simulink model "SDA_PL_Harness_2025b"  (R2025b)
settings: Solver=FixedStepDiscrete  StartTime=0.0  StopTime=inf  FixedStep=1e-8  RelTol=1e-3
PreLoadFcn:
  | addpath('C:\Users\Cheng\Documents\MasterThesis\Model_2025b\Harness');
InitFcn:
  | setup_sda_harness_workspace_2025b;
undefined symbols (not defined in the file or in its folder): sdaHarnessAbsTol, sdaHarnessCaseLimit, sdaHarnessData, sdaHarnessRelTol
(part 1 of 2)
settings Model: DataDictionary=FOC_params.sldd  Creator=Cheng  LastModifiedBy=Cheng

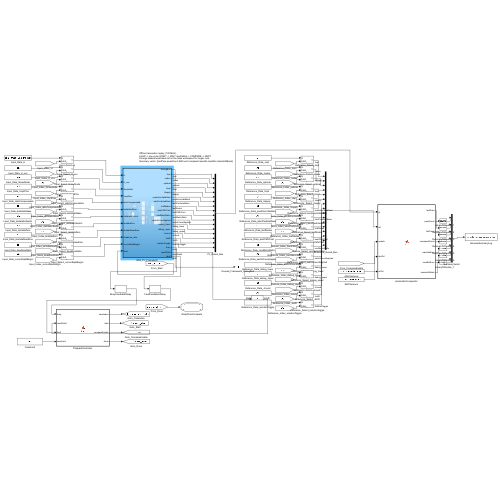
[thumbnail: Simulink's stored preview of the top-level diagram]
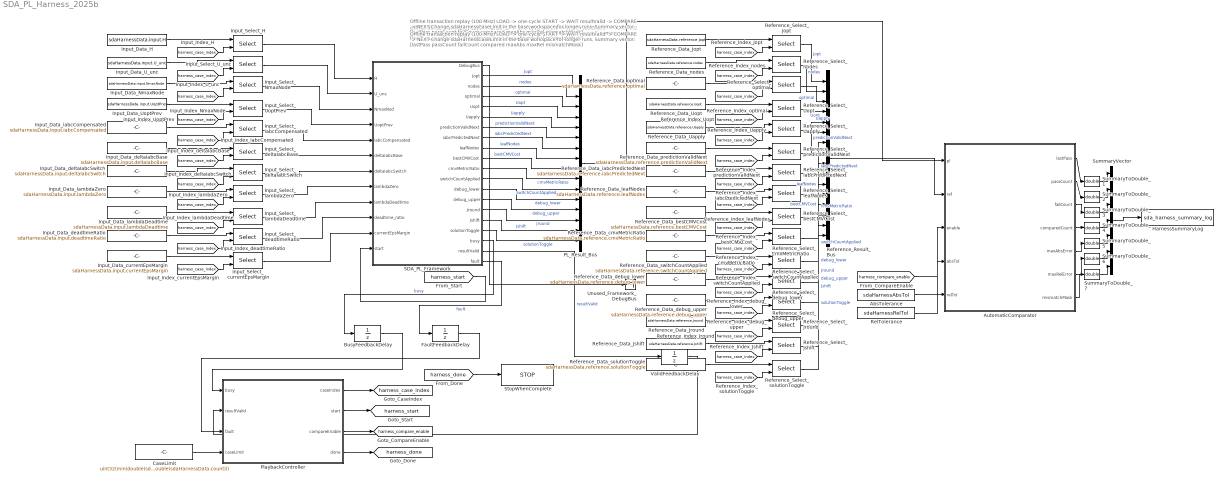
== system SDA_PL_Harness_2025b ==
  note: Offline transaction replay (100 MHz)
      | LOAD -> one-cycle START -> WAIT resultValid -> COMPARE -> NEXT
      | Change sdaHarnessCaseLimit in the base workspace for longer runs.
      | Summary vector: [lastPass passCount failCount compared maxAbs maxRel mismatchMask]
  note: Offline transaction replay (100 MHz)
      | LOAD -> one-cycle START -> WAIT resultValid -> COMPARE -> NEXT
      | Change sdaHarnessCaseLimit in the base workspace for longer runs.
      | Summary vector: [lastPass passCount failCount compared maxAbs maxRel mismatchMask]
  note: Offline transaction replay (100 MHz)
      | LOAD -> one-cycle START -> WAIT resultValid -> COMPARE -> NEXT
      | Change sdaHarnessCaseLimit in the base workspace for longer runs.
      | Summary vector: [lastPass passCount failCount compared maxAbs maxRel mismatchMask]
  note: Offline transaction replay (100 MHz)
      | LOAD -> one-cycle START -> WAIT resultValid -> COMPARE -> NEXT
      | Change sdaHarnessCaseLimit in the base workspace for longer runs.
      | Summary vector: [lastPass passCount failCount compared maxAbs maxRel mismatchMask]
  note: Offline transaction replay (100 MHz)
      | LOAD -> one-cycle START -> WAIT resultValid -> COMPARE -> NEXT
      | Change sdaHarnessCaseLimit in the base workspace for longer runs.
      | Summary vector: [lastPass passCount failCount compared maxAbs maxRel mismatchMask]
  note: Offline transaction replay (100 MHz)
      | LOAD -> one-cycle START -> WAIT resultValid -> COMPARE -> NEXT
      | Change sdaHarnessCaseLimit in the base workspace for longer runs.
      | Summary vector: [lastPass passCount failCount compared maxAbs maxRel mismatchMask]
  AbsTolerance : Constant  Value=sdaHarnessAbsTol
  AutomaticComparator : MATLAB Function  TreatAsAtomicUnit=on
  BusyFeedbackDelay : UnitDelay  InitialCondition=false  SampleTime=1e-8  HasFrameUpgradeWarning=on
  CaseLimit : Constant  Value=uint32(min(double(sdaHarnessCaseLimit),double(sdaHarnessData.count)))  OutDataTypeStr=uint32
  FaultFeedbackDelay : UnitDelay  InitialCondition=false  SampleTime=1e-8  HasFrameUpgradeWarning=on
  HarnessSummaryLog : ToWorkspace  VariableName=sda_harness_summary_log  SaveFormat=Timeseries  SampleTime=-1
  Input_Data_H : Constant  Value=sdaHarnessData.input.H
  Input_Data_NmaxNode : Constant  Value=sdaHarnessData.input.NmaxNode
  Input_Data_U_unc : Constant  Value=sdaHarnessData.input.U_unc
  Input_Data_UoptPrev : Constant  Value=sdaHarnessData.input.UoptPrev
  Input_Data_currentEpsMargin : Constant  Value=sdaHarnessData.input.currentEpsMargin
  Input_Data_deadtimeRatio : Constant  Value=sdaHarnessData.input.deadtimeRatio
  Input_Data_deltaIabcBase : Constant  Value=sdaHarnessData.input.deltaIabcBase
  Input_Data_deltaIabcSwitch : Constant  Value=sdaHarnessData.input.deltaIabcSwitch
  Input_Data_iabcCompensated : Constant  Value=sdaHarnessData.input.iabcCompensated
  Input_Data_lambdaDeadtime : Constant  Value=sdaHarnessData.input.lambdaDeadtime
  Input_Data_lambdaZero : Constant  Value=sdaHarnessData.input.lambdaZero
  Input_Select_H : Selector  NumberOfDimensions=3  InputPortWidth=3  IndexOptions=Select all,Select all,Index vector (port)  Indices=1,1,1  OutputSizes=1
  Input_Select_NmaxNode : Selector  NumberOfDimensions=2  InputPortWidth=3  IndexOptions=Index vector (dialog),Index vector (port)  Indices=1,1  OutputSizes=1
  Input_Select_U_unc : Selector  NumberOfDimensions=2  InputPortWidth=3  IndexOptions=Select all,Index vector (port)  Indices=1,1  OutputSizes=1
  Input_Select_UoptPrev : Selector  NumberOfDimensions=2  InputPortWidth=3  IndexOptions=Select all,Index vector (port)  Indices=1,1  OutputSizes=1
  Input_Select_currentEpsMargin : Selector  NumberOfDimensions=2  InputPortWidth=3  IndexOptions=Index vector (dialog),Index vector (port)  Indices=1,1  OutputSizes=1
  Input_Select_deadtimeRatio : Selector  NumberOfDimensions=2  InputPortWidth=3  IndexOptions=Index vector (dialog),Index vector (port)  Indices=1,1  OutputSizes=1
  Input_Select_deltaIabcBase : Selector  NumberOfDimensions=2  InputPortWidth=3  IndexOptions=Select all,Index vector (port)  Indices=1,1  OutputSizes=1
  Input_Select_deltaIabcSwitch : Selector  NumberOfDimensions=3  InputPortWidth=3  IndexOptions=Select all,Select all,Index vector (port)  Indices=1,1,1  OutputSizes=1
  Input_Select_iabcCompensated : Selector  NumberOfDimensions=2  InputPortWidth=3  IndexOptions=Select all,Index vector (port)  Indices=1,1  OutputSizes=1
  Input_Select_lambdaDeadtime : Selector  NumberOfDimensions=2  InputPortWidth=3  IndexOptions=Index vector (dialog),Index vector (port)  Indices=1,1  OutputSizes=1
  Input_Select_lambdaZero : Selector  NumberOfDimensions=2  InputPortWidth=3  IndexOptions=Index vector (dialog),Index vector (port)  Indices=1,1  OutputSizes=1
  PL_Result_Bus : BusCreator  Inputs=16  OutDataTypeStr=Bus: SdaComparisonResultBus
  PlaybackController : MATLAB Function  TreatAsAtomicUnit=on
  Reference_Data_Jopt : Constant  Value=sdaHarnessData.reference.Jopt
  Reference_Data_Jround : Constant  Value=sdaHarnessData.reference.Jround
  Reference_Data_Jshift : Constant  Value=sdaHarnessData.reference.Jshift
  Reference_Data_Uapply : Constant  Value=sdaHarnessData.reference.Uapply
  Reference_Data_Uopt : Constant  Value=sdaHarnessData.reference.Uopt
  Reference_Data_bestCMVCost : Constant  Value=sdaHarnessData.reference.bestCMVCost
  Reference_Data_cmvMetricRatio : Constant  Value=sdaHarnessData.reference.cmvMetricRatio
  Reference_Data_debug_lower : Constant  Value=sdaHarnessData.reference.debug_lower
  Reference_Data_debug_upper : Constant  Value=sdaHarnessData.reference.debug_upper
  Reference_Data_iabcPredictedNext : Constant  Value=sdaHarnessData.reference.iabcPredictedNext
  Reference_Data_leafNodes : Constant  Value=sdaHarnessData.reference.leafNodes
  Reference_Data_nodes : Constant  Value=sdaHarnessData.reference.nodes
  Reference_Data_optimal : Constant  Value=sdaHarnessData.reference.optimal
  Reference_Data_predictionValidNext : Constant  Value=sdaHarnessData.reference.predictionValidNext
  Reference_Data_solutionToggle : Constant  Value=sdaHarnessData.reference.solutionToggle
  Reference_Data_switchCountApplied : Constant  Value=sdaHarnessData.reference.switchCountApplied
  Reference_Result_Bus : BusCreator  Inputs=16  OutDataTypeStr=Bus: SdaComparisonResultBus
  Reference_Select_Jopt : Selector  NumberOfDimensions=2  InputPortWidth=3  IndexOptions=Index vector (dialog),Index vector (port)  Indices=1,1  OutputSizes=1
  Reference_Select_Jround : Selector  NumberOfDimensions=2  InputPortWidth=3  IndexOptions=Index vector (dialog),Index vector (port)  Indices=1,1  OutputSizes=1
  Reference_Select_Jshift : Selector  NumberOfDimensions=2  InputPortWidth=3  IndexOptions=Index vector (dialog),Index vector (port)  Indices=1,1  OutputSizes=1
  Reference_Select_Uapply : Selector  NumberOfDimensions=2  InputPortWidth=3  IndexOptions=Select all,Index vector (port)  Indices=1,1  OutputSizes=1
  Reference_Select_Uopt : Selector  NumberOfDimensions=2  InputPortWidth=3  IndexOptions=Select all,Index vector (port)  Indices=1,1  OutputSizes=1
  Reference_Select_bestCMVCost : Selector  NumberOfDimensions=2  InputPortWidth=3  IndexOptions=Index vector (dialog),Index vector (port)  Indices=1,1  OutputSizes=1
  Reference_Select_cmvMetricRatio : Selector  NumberOfDimensions=2  InputPortWidth=3  IndexOptions=Index vector (dialog),Index vector (port)  Indices=1,1  OutputSizes=1
  Reference_Select_debug_lower : Selector  NumberOfDimensions=2  InputPortWidth=3  IndexOptions=Select all,Index vector (port)  Indices=1,1  OutputSizes=1
  Reference_Select_debug_upper : Selector  NumberOfDimensions=2  InputPortWidth=3  IndexOptions=Select all,Index vector (port)  Indices=1,1  OutputSizes=1
  Reference_Select_iabcPredictedNext : Selector  NumberOfDimensions=2  InputPortWidth=3  IndexOptions=Select all,Index vector (port)  Indices=1,1  OutputSizes=1
  Reference_Select_leafNodes : Selector  NumberOfDimensions=2  InputPortWidth=3  IndexOptions=Index vector (dialog),Index vector (port)  Indices=1,1  OutputSizes=1
  Reference_Select_nodes : Selector  NumberOfDimensions=2  InputPortWidth=3  IndexOptions=Index vector (dialog),Index vector (port)  Indices=1,1  OutputSizes=1
  Reference_Select_optimal : Selector  NumberOfDimensions=2  InputPortWidth=3  IndexOptions=Index vector (dialog),Index vector (port)  Indices=1,1  OutputSizes=1
  Reference_Select_predictionValidNext : Selector  NumberOfDimensions=2  InputPortWidth=3  IndexOptions=Index vector (dialog),Index vector (port)  Indices=1,1  OutputSizes=1
  Reference_Select_solutionToggle : Selector  NumberOfDimensions=2  InputPortWidth=3  IndexOptions=Index vector (dialog),Index vector (port)  Indices=1,1  OutputSizes=1
  Reference_Select_switchCountApplied : Selector  NumberOfDimensions=2  InputPortWidth=3  IndexOptions=Index vector (dialog),Index vector (port)  Indices=1,1  OutputSizes=1
  RelTolerance : Constant  Value=sdaHarnessRelTol
  SDA_PL_Framework : Subsystem  TreatAsAtomicUnit=on
  StopWhenComplete : Stop
  SummaryToDouble_{1..7} (7 alike) : DataTypeConversion  OutDataTypeStr=double  SaturateOnIntegerOverflow=off  RndMeth=Floor
  SummaryVector : Mux  Inputs=7
  Unused_Framework_DebugBus : Terminator
  ValidFeedbackDelay : UnitDelay  InitialCondition=false  SampleTime=1e-8  HasFrameUpgradeWarning=on
  tag scope: harness_case_index=global, harness_compare_enable=global, harness_done=global, harness_start=global
  wires:
  CaseLimit/1 -> PlaybackController/4(caseLimit)
  PlaybackController/1(caseIndex) -> [harness_case_index]
  PlaybackController/2(start) -> [harness_start]
  PlaybackController/3(compareEnable) -> [harness_compare_enable]
  PlaybackController/4(done) -> [harness_done]
  Input_Data_H/1 -> Input_Select_H/1
  [harness_case_index] -> Input_Select_H/2
  Input_Data_U_unc/1 -> Input_Select_U_unc/1
  [harness_case_index] -> Input_Select_U_unc/2
  Input_Data_NmaxNode/1 -> Input_Select_NmaxNode/1
  [harness_case_index] -> Input_Select_NmaxNode/2
  Input_Data_UoptPrev/1 -> Input_Select_UoptPrev/1
  [harness_case_index] -> Input_Select_UoptPrev/2
  Input_Data_iabcCompensated/1 -> Input_Select_iabcCompensated/1
  [harness_case_index] -> Input_Select_iabcCompensated/2
  Input_Data_deltaIabcBase/1 -> Input_Select_deltaIabcBase/1
  [harness_case_index] -> Input_Select_deltaIabcBase/2
  Input_Data_deltaIabcSwitch/1 -> Input_Select_deltaIabcSwitch/1
  [harness_case_index] -> Input_Select_deltaIabcSwitch/2
  Input_Data_lambdaZero/1 -> Input_Select_lambdaZero/1
  [harness_case_index] -> Input_Select_lambdaZero/2
  Input_Data_lambdaDeadtime/1 -> Input_Select_lambdaDeadtime/1
  [harness_case_index] -> Input_Select_lambdaDeadtime/2
  Input_Data_deadtimeRatio/1 -> Input_Select_deadtimeRatio/1
  [harness_case_index] -> Input_Select_deadtimeRatio/2
  Input_Data_currentEpsMargin/1 -> Input_Select_currentEpsMargin/1
  [harness_case_index] -> Input_Select_currentEpsMargin/2
  Reference_Data_Jopt/1 -> Reference_Select_Jopt/1
  [harness_case_index] -> Reference_Select_Jopt/2
  Reference_Data_nodes/1 -> Reference_Select_nodes/1
  [harness_case_index] -> Reference_Select_nodes/2
  Reference_Data_optimal/1 -> Reference_Select_optimal/1
  [harness_case_index] -> Reference_Select_optimal/2
  Reference_Data_Uopt/1 -> Reference_Select_Uopt/1
  [harness_case_index] -> Reference_Select_Uopt/2
  Reference_Data_Uapply/1 -> Reference_Select_Uapply/1
  [harness_case_index] -> Reference_Select_Uapply/2
  Reference_Data_predictionValidNext/1 -> Reference_Select_predictionValidNext/1
  [harness_case_index] -> Reference_Select_predictionValidNext/2
  Reference_Data_iabcPredictedNext/1 -> Reference_Select_iabcPredictedNext/1
  [harness_case_index] -> Reference_Select_iabcPredictedNext/2
  Reference_Data_leafNodes/1 -> Reference_Select_leafNodes/1
  [harness_case_index] -> Reference_Select_leafNodes/2
  Reference_Data_bestCMVCost/1 -> Reference_Select_bestCMVCost/1
  [harness_case_index] -> Reference_Select_bestCMVCost/2
  Reference_Data_cmvMetricRatio/1 -> Reference_Select_cmvMetricRatio/1
  [harness_case_index] -> Reference_Select_cmvMetricRatio/2
  Reference_Data_switchCountApplied/1 -> Reference_Select_switchCountApplied/1
  [harness_case_index] -> Reference_Select_switchCountApplied/2
  Reference_Data_debug_lower/1 -> Reference_Select_debug_lower/1
  [harness_case_index] -> Reference_Select_debug_lower/2
  Reference_Data_debug_upper/1 -> Reference_Select_debug_upper/1
  [harness_case_index] -> Reference_Select_debug_upper/2
  Reference_Data_Jround/1 -> Reference_Select_Jround/1
  [harness_case_index] -> Reference_Select_Jround/2
  Reference_Data_Jshift/1 -> Reference_Select_Jshift/1
  [harness_case_index] -> Reference_Select_Jshift/2
  Reference_Data_solutionToggle/1 -> Reference_Select_solutionToggle/1
  [harness_case_index] -> Reference_Select_solutionToggle/2
  Input_Select_H/1 -> SDA_PL_Framework/1(H)
  Input_Select_U_unc/1 -> SDA_PL_Framework/2(U_unc)
  Input_Select_NmaxNode/1 -> SDA_PL_Framework/3(NmaxNod)
  Input_Select_UoptPrev/1 -> SDA_PL_Framework/4(UoptPrev)
  Input_Select_iabcCompensated/1 -> SDA_PL_Framework/5(iabcCompensated)
  Input_Select_deltaIabcBase/1 -> SDA_PL_Framework/6(deltaIabcBase)
  Input_Select_deltaIabcSwitch/1 -> SDA_PL_Framework/7(deltaIabcSwitch)
  Input_Select_lambdaZero/1 -> SDA_PL_Framework/8(lambdaZero)
  Input_Select_lambdaDeadtime/1 -> SDA_PL_Framework/9(lambdaDeadtime)
  Input_Select_deadtimeRatio/1 -> SDA_PL_Framework/10(deadtime_ratio)
  Input_Select_currentEpsMargin/1 -> SDA_PL_Framework/11(currentEpsMargin)
  [harness_start] -> SDA_PL_Framework/12(start)
  SDA_PL_Framework/2(Jopt) -> PL_Result_Bus/1  "Jopt"
  Reference_Select_Jopt/1 -> Reference_Result_Bus/1  "Jopt"
  SDA_PL_Framework/3(nodes) -> PL_Result_Bus/2  "nodes"
  Reference_Select_nodes/1 -> Reference_Result_Bus/2  "nodes"
  SDA_PL_Framework/4(optimal) -> PL_Result_Bus/3  "optimal"
  Reference_Select_optimal/1 -> Reference_Result_Bus/3  "optimal"
  SDA_PL_Framework/5(Uopt) -> PL_Result_Bus/4  "Uopt"
  Reference_Select_Uopt/1 -> Reference_Result_Bus/4  "Uopt"
  SDA_PL_Framework/6(Uapply) -> PL_Result_Bus/5  "Uapply"
  Reference_Select_Uapply/1 -> Reference_Result_Bus/5  "Uapply"
  SDA_PL_Framework/7(predictionValidNext) -> PL_Result_Bus/6  "predictionValidNext"
  Reference_Select_predictionValidNext/1 -> Reference_Result_Bus/6  "predictionValidNext"
  SDA_PL_Framework/8(iabcPredictedNext) -> PL_Result_Bus/7  "iabcPredictedNext"
  Reference_Select_iabcPredictedNext/1 -> Reference_Result_Bus/7  "iabcPredictedNext"
  SDA_PL_Framework/9(leafNodes) -> PL_Result_Bus/8  "leafNodes"
  Reference_Select_leafNodes/1 -> Reference_Result_Bus/8  "leafNodes"
  SDA_PL_Framework/10(bestCMVCost) -> PL_Result_Bus/9  "bestCMVCost"
  Reference_Select_bestCMVCost/1 -> Reference_Result_Bus/9  "bestCMVCost"
  SDA_PL_Framework/11(cmvMetricRatio) -> PL_Result_Bus/10  "cmvMetricRatio"
  Reference_Select_cmvMetricRatio/1 -> Reference_Result_Bus/10  "cmvMetricRatio"
  SDA_PL_Framework/12(switchCountApplied) -> PL_Result_Bus/11  "switchCountApplied"
  Reference_Select_switchCountApplied/1 -> Reference_Result_Bus/11  "switchCountApplied"
  SDA_PL_Framework/13(debug_lower) -> PL_Result_Bus/12  "debug_lower"
  Reference_Select_debug_lower/1 -> Reference_Result_Bus/12  "debug_lower"
  SDA_PL_Framework/14(debug_upper) -> PL_Result_Bus/13  "debug_upper"
  Reference_Select_debug_upper/1 -> Reference_Result_Bus/13  "debug_upper"
  SDA_PL_Framework/15(Jround) -> PL_Result_Bus/14  "Jround"
  Reference_Select_Jround/1 -> Reference_Result_Bus/14  "Jround"
  SDA_PL_Framework/16(Jshift) -> PL_Result_Bus/15  "Jshift"
  Reference_Select_Jshift/1 -> Reference_Result_Bus/15  "Jshift"
  SDA_PL_Framework/17(solutionToggle) -> PL_Result_Bus/16  "solutionToggle"
  Reference_Select_solutionToggle/1 -> Reference_Result_Bus/16  "solutionToggle"
  PL_Result_Bus/1 -> AutomaticComparator/1(pl)
  Reference_Result_Bus/1 -> AutomaticComparator/2(ref)
  [harness_compare_enable] -> AutomaticComparator/3(enable)
  AbsTolerance/1 -> AutomaticComparator/4(absTol)
  RelTolerance/1 -> AutomaticComparator/5(relTol)
  AutomaticComparator/1(lastPass) -> SummaryToDouble_1/1
  SummaryToDouble_1/1 -> SummaryVector/1
  AutomaticComparator/2(passCount) -> SummaryToDouble_2/1
  SummaryToDouble_2/1 -> SummaryVector/2
  AutomaticComparator/3(failCount) -> SummaryToDouble_3/1
  SummaryToDouble_3/1 -> SummaryVector/3
  AutomaticComparator/4(comparedCount) -> SummaryToDouble_4/1
  SummaryToDouble_4/1 -> SummaryVector/4
  AutomaticComparator/5(maxAbsError) -> SummaryToDouble_5/1
  SummaryToDouble_5/1 -> SummaryVector/5
  AutomaticComparator/6(maxRelError) -> SummaryToDouble_6/1
  SummaryToDouble_6/1 -> SummaryVector/6
  AutomaticComparator/7(mismatchMask) -> SummaryToDouble_7/1
  SummaryToDouble_7/1 -> SummaryVector/7
  SummaryVector/1 -> HarnessSummaryLog/1
  [harness_done] -> StopWhenComplete/1
  SDA_PL_Framework/18(busy) -> BusyFeedbackDelay/1  "busy"
  BusyFeedbackDelay/1 -> PlaybackController/1(busy)
  SDA_PL_Framework/19(resultValid) -> ValidFeedbackDelay/1  "resultValid"
  ValidFeedbackDelay/1 -> PlaybackController/2(resultValid)
  SDA_PL_Framework/20(fault) -> FaultFeedbackDelay/1  "fault"
  FaultFeedbackDelay/1 -> PlaybackController/3(fault)
  SDA_PL_Framework/1(DebugBus) -> Unused_Framework_DebugBus/1

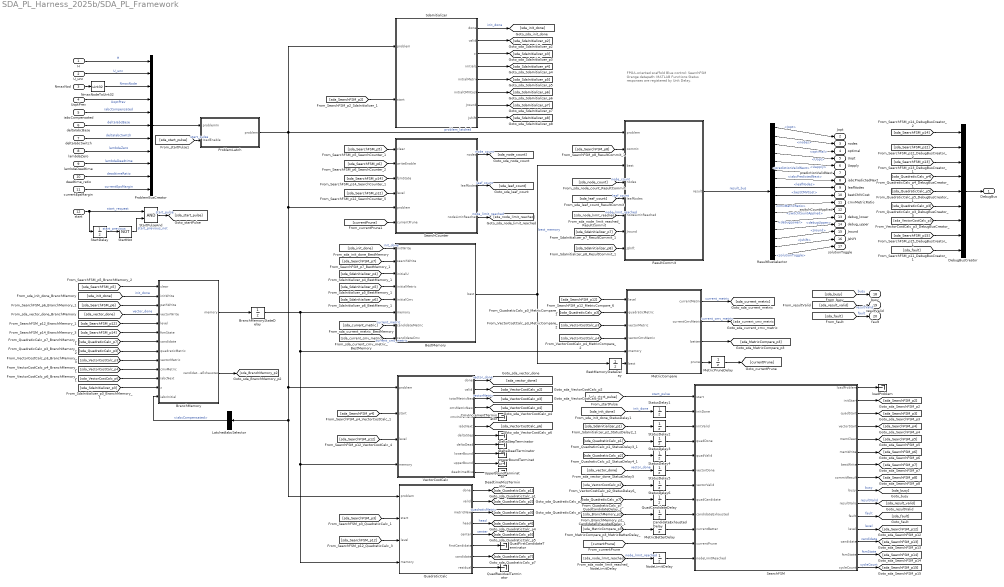
== system SDA_PL_Harness_2025b/SDA_PL_Framework ==
  note: FPGA-oriented scaffold
      | Blue control: SearchFSM
      | Orange datapath: MATLAB Functions
      | Status responses are registered by Unit Delay.
  H : Inport
  U_unc : Inport  Port=2
  NmaxNod : Inport  Port=3
  UoptPrev : Inport  Port=4
  iabcCompensated : Inport  Port=5
  deltaIabcBase : Inport  Port=6
  deltaIabcSwitch : Inport  Port=7
  lambdaZero : Inport  Port=8
  lambdaDeadtime : Inport  Port=9
  deadtime_ratio : Inport  Port=10
  currentEpsMargin : Inport  Port=11
  start : Inport  Port=12  OutDataTypeStr=boolean
  BestMemory : MATLAB Function  TreatAsAtomicUnit=on
  BestMemoryStateDelay : UnitDelay  SampleTime=-1
  BranchMemory : MATLAB Function  TreatAsAtomicUnit=on
  BranchMemoryStateDelay : UnitDelay  SampleTime=-1
  CandidateExhaustedDelay : UnitDelay  InitialCondition=false  SampleTime=-1
  CmvIncrementTerminator : Terminator
  DeadtimeMissTerminator : Terminator
  DebugBusCreator : BusCreator  Inputs=9  OutDataTypeStr=Bus: SdaDebugBus
  DeltaDeadTerminator : Terminator
  DeltaStepTerminator : Terminator
  LatchedIabcSelector : BusSelector  OutputSignals=iabcCompensated
  LowerBoundTerminator : Terminator
  MetricBetterDelay : UnitDelay  InitialCondition=false  SampleTime=-1
  MetricCompare : MATLAB Function  TreatAsAtomicUnit=on
  MetricPruneDelay : UnitDelay  InitialCondition=false  SampleTime=-1
  NmaxNodeToUint32 : DataTypeConversion  OutDataTypeStr=uint32  SaturateOnIntegerOverflow=off  RndMeth=Floor
  NodeLimitDelay : UnitDelay  InitialCondition=false  SampleTime=-1
  ProblemBusCreator : BusCreator  Inputs=11  OutDataTypeStr=Bus: SdaProblemBus
  ProblemLatch : MATLAB Function  TreatAsAtomicUnit=on
  QuadCandidateDelay : UnitDelay  InitialCondition=false  SampleTime=-1
  QuadFirstCandidateTerminator : Terminator
  QuadResidualTerminator : Terminator
  QuadraticCalc : MATLAB Function  TreatAsAtomicUnit=on
  ResultBusSelector : BusSelector  OutputSignals=Jopt,nodes,optimal,Uopt,Uapply,predictionValidNext,iabcPredictedNext,leafNodes,bestCMVCost,cmvMetricRatio,switchCountApplied,debugLower,debugUpper,Jround,Jshift,solutionToggle
  ResultCommit : MATLAB Function  TreatAsAtomicUnit=on
  SdaInitializer : MATLAB Function  TreatAsAtomicUnit=on
  SearchCounter : MATLAB Function  TreatAsAtomicUnit=on
  SearchFSM : Stateflow chart  TreatAsAtomicUnit=on
  StartDelay : UnitDelay  InitialCondition=false  SampleTime=-1  HasFrameUpgradeWarning=on
  StartNot : Logic  Operator=NOT  AllPortsSameDT=off  OutDataTypeStr=boolean
  StartPulseAnd : Logic  AllPortsSameDT=off  OutDataTypeStr=boolean
  StatusDelay{1..6} (6 alike) : UnitDelay  InitialCondition=false  SampleTime=-1
  UpperBoundTerminator : Terminator
  VectorCostCalc : MATLAB Function  TreatAsAtomicUnit=on
  loadProblem : Terminator
  DebugBus : Outport  OutDataTypeStr=Bus: SdaDebugBus
  Jopt : Outport  Port=2
  nodes : Outport  Port=3
  optimal : Outport  Port=4
  Uopt : Outport  Port=5
  Uapply : Outport  Port=6
  predictionValidNext : Outport  Port=7
  iabcPredictedNext : Outport  Port=8
  leafNodes : Outport  Port=9
  bestCMVCost : Outport  Port=10
  cmvMetricRatio : Outport  Port=11
  switchCountApplied : Outport  Port=12
  debug_lower : Outport  Port=13
  debug_upper : Outport  Port=14
  Jround : Outport  Port=15
  Jshift : Outport  Port=16
  solutionToggle : Outport  Port=17
  busy : Outport  Port=18
  resultValid : Outport  Port=19
  fault : Outport  Port=20
  wires:
  NodeLimitDelay/1 -> SearchFSM/12(nodeLimitReached)
  MetricPruneDelay/1 -> [currentPrune]
  MetricBetterDelay/1 -> SearchFSM/10(currentBetter)
  BestMemoryStateDelay/1 -> MetricCompare/6(best)
  CandidateExhaustedDelay/1 -> SearchFSM/9(candidateExhausted)
  QuadCandidateDelay/1 -> SearchFSM/8(quadCandidate)
  BranchMemoryStateDelay/1 -> QuadraticCalc/4(memory), VectorCostCalc/4(memory), MetricCompare/5(memory), BestMemory/6(memory)
  NmaxNodeToUint32/1 -> ProblemBusCreator/3  "NmaxNode"
  NmaxNod/1 -> NmaxNodeToUint32/1
  DebugBusCreator/1 -> DebugBus/1
  SearchFSM/11(fault) -> [sda_fault]  "fault"
  StatusDelay6/1 -> SearchFSM/7(vectorValid)
  StatusDelay5/1 -> SearchFSM/6(vectorDone)
  StatusDelay4/1 -> SearchFSM/5(quadValid)
  StatusDelay3/1 -> SearchFSM/4(quadDone)
  StatusDelay2/1 -> SearchFSM/3(initValid)
  StatusDelay1/1 -> SearchFSM/2(initDone)
  ProblemBusCreator/1 -> ProblemLatch/1(problemIn)
  currentEpsMargin/1 -> ProblemBusCreator/11  "currentEpsMargin"
  deadtime_ratio/1 -> ProblemBusCreator/10  "deadtimeRatio"
  lambdaDeadtime/1 -> ProblemBusCreator/9  "lambdaDeadtime"
  lambdaZero/1 -> ProblemBusCreator/8  "lambdaZero"
  deltaIabcSwitch/1 -> ProblemBusCreator/7  "deltaIabcSwitch"
  deltaIabcBase/1 -> ProblemBusCreator/6  "deltaIabcBase"
  iabcCompensated/1 -> ProblemBusCreator/5  "iabcCompensated"
  UoptPrev/1 -> ProblemBusCreator/4  "UoptPrev"
  U_unc/1 -> ProblemBusCreator/2  "U_unc"
  H/1 -> ProblemBusCreator/1  "H"
  start/1 -> StartDelay/1, StartPulseAnd/1  "start_request"
  StartDelay/1 -> StartNot/1  "start_previous"
  StartNot/1 -> StartPulseAnd/2  "start_previous_not"
  StartPulseAnd/1 -> [sda_start_pulse]  "start_pulse"
  [sda_start_pulse] -> SearchFSM/1(start)  "start_pulse"
  ResultBusSelector/1 -> Jopt/1  "<Jopt>"
  ResultBusSelector/2 -> nodes/1  "<nodes>"
  ResultBusSelector/3 -> optimal/1  "<optimal>"
  ResultBusSelector/4 -> Uopt/1  "<Uopt>"
  ResultBusSelector/5 -> Uapply/1  "<Uapply>"
  ResultBusSelector/6 -> predictionValidNext/1  "<predictionValidNext>"
  ResultBusSelector/7 -> iabcPredictedNext/1  "<iabcPredictedNext>"
  ResultBusSelector/8 -> leafNodes/1  "<leafNodes>"
  ResultBusSelector/9 -> bestCMVCost/1  "<bestCMVCost>"
  ResultBusSelector/10 -> cmvMetricRatio/1  "<cmvMetricRatio>"
  ResultBusSelector/11 -> switchCountApplied/1  "<switchCountApplied>"
  ResultBusSelector/12 -> debug_lower/1  "<debugLower>"
  ResultBusSelector/13 -> debug_upper/1  "<debugUpper>"
  ResultBusSelector/14 -> Jround/1  "<Jround>"
  ResultBusSelector/15 -> Jshift/1  "<Jshift>"
  ResultBusSelector/16 -> solutionToggle/1  "<solutionToggle>"
  SearchFSM/9(busy) -> [sda_busy]  "busy"
  [sda_busy] -> busy/1  "busy"
  SearchFSM/10(resultValid) -> [sda_result_valid]  "resultValid"
  [sda_result_valid] -> resultValid/1  "resultValid"
  [sda_fault] -> fault/1  "fault"
  ProblemLatch/1(problem) -> QuadraticCalc/1(problem), LatchedIabcSelector/1, VectorCostCalc/1(problem), SearchCounter/5(problem), ResultCommit/1(problem), SdaInitializer/1(problem)  "problem_latched"
  BestMemory/1(best) -> ResultCommit/3(best), BestMemoryStateDelay/1  "best_memory"
  ResultCommit/1(result) -> ResultBusSelector/1  "result_bus"
  SdaInitializer/1(done) -> [sda_init_done]  "init_done"
  [sda_init_done] -> StatusDelay1/1  "init_done"
  [sda_init_done] -> BranchMemory/2(initWrite)  "init_done"
  [sda_init_done] -> BestMemory/1(initWrite)  "init_done"
  VectorCostCalc/1(done) -> [sda_vector_done]  "vector_done"
  [sda_vector_done] -> BranchMemory/4(vectorWrite)  "vector_done"
  [sda_vector_done] -> StatusDelay5/1  "vector_done"
  MetricCompare/1(currentMetric) -> [sda_current_metric]  "current_metric"
  [sda_current_metric] -> BestMemory/7(candidateMetric)  "current_metric"
  MetricCompare/2(currentCmvMetric) -> [sda_current_cmv_metric]  "current_cmv_metric"
  [sda_current_cmv_metric] -> BestMemory/8(candidateCmv)  "current_cmv_metric"
  SearchCounter/1(nodes) -> [sda_node_count]  "node_count"
  [sda_node_count] -> ResultCommit/4(nodes)  "node_count"
  SearchCounter/2(leafNodes) -> [sda_leaf_count]  "leaf_count"
  [sda_leaf_count] -> ResultCommit/5(leafNodes)  "leaf_count"
  SearchCounter/3(nodeLimitReached) -> [sda_node_limit_reached]  "node_limit_reached"
  [sda_node_limit_reached] -> ResultCommit/6(nodeLimitReached)  "node_limit_reached"
  [sda_node_limit_reached] -> NodeLimitDelay/1  "node_limit_reached"
  SearchFSM/1(loadProblem) -> loadProblem/1
  SearchFSM/2(initStart) -> [sda_SearchFSM_p2]
  [sda_SearchFSM_p2] -> SdaInitializer/2(start)
  SearchFSM/3(quadStart) -> [sda_SearchFSM_p3]
  [sda_SearchFSM_p3] -> QuadraticCalc/2(start)
  SearchFSM/4(vectorStart) -> [sda_SearchFSM_p4]
  [sda_SearchFSM_p4] -> VectorCostCalc/2(start)
  SearchFSM/5(memClear) -> [sda_SearchFSM_p5]
  [sda_SearchFSM_p5] -> SearchCounter/1(clear)
  [sda_SearchFSM_p5] -> BranchMemory/1(clear)
  SearchFSM/6(memWrite) -> [sda_SearchFSM_p6]
  [sda_SearchFSM_p6] -> BranchMemory/3(pathWrite)
  [sda_SearchFSM_p6] -> SearchCounter/2(writeEnable)
  SearchFSM/7(bestWrite) -> [sda_SearchFSM_p7]
  [sda_SearchFSM_p7] -> BestMemory/2(searchWrite)
  SearchFSM/8(commitResult) -> [sda_SearchFSM_p8]
  [sda_SearchFSM_p8] -> ResultCommit/2(commit)
  [sda_fault] -> DebugBusCreator/9
  SearchFSM/12(level) -> [sda_SearchFSM_p12]  "level"
  [sda_SearchFSM_p12] -> BranchMemory/5(level)
  [sda_SearchFSM_p12] -> DebugBusCreator/2
  [sda_SearchFSM_p12] -> QuadraticCalc/3(level)
  [sda_SearchFSM_p12] -> VectorCostCalc/3(level)
  [sda_SearchFSM_p12] -> SearchCounter/4(level)
  [sda_SearchFSM_p12] -> MetricCompare/1(level)
  SearchFSM/13(candidate) -> [sda_SearchFSM_p13]  "candidate"
  [sda_SearchFSM_p13] -> DebugBusCreator/3
  SearchFSM/14(fsmState) -> [sda_SearchFSM_p14]  "fsmState"
  [sda_SearchFSM_p14] -> SearchCounter/3(fsmState)
  [sda_SearchFSM_p14] -> DebugBusCreator/1
  [sda_SearchFSM_p14] -> BranchMemory/6(fsmState)
  SearchFSM/15(cycleCount) -> [sda_SearchFSM_p15]  "cycleCount"
  [sda_SearchFSM_p15] -> DebugBusCreator/8
  SdaInitializer/2(valid) -> [sda_SdaInitializer_p2]
  [sda_SdaInitializer_p2] -> StatusDelay2/1
  SdaInitializer/3(z) -> [sda_SdaInitializer_p3]
  [sda_SdaInitializer_p3] -> BranchMemory/12(z)
  SdaInitializer/4(initialU) -> [sda_SdaInitializer_p4]
  [sda_SdaInitializer_p4] -> BestMemory/3(initialU)
  SdaInitializer/5(initialMetric) -> [sda_SdaInitializer_p5]
  [sda_SdaInitializer_p5] -> BestMemory/4(initialMetric)
  SdaInitializer/6(initialCMVCost) -> [sda_SdaInitializer_p6]
  [sda_SdaInitializer_p6] -> BestMemory/5(initialCmv)
  SdaInitializer/7(Jround) -> [sda_SdaInitializer_p7]
  [sda_SdaInitializer_p7] -> ResultCommit/7(Jround)
  SdaInitializer/8(Jshift) -> [sda_SdaInitializer_p8]
  [sda_SdaInitializer_p8] -> ResultCommit/8(Jshift)
  QuadraticCalc/1(done) -> [sda_QuadraticCalc_p1]
  [sda_QuadraticCalc_p1] -> StatusDelay3/1
  QuadraticCalc/2(valid) -> [sda_QuadraticCalc_p2]
  [sda_QuadraticCalc_p2] -> StatusDelay4/1
  QuadraticCalc/3(metricNew) -> [sda_QuadraticCalc_p3]  "quadraticMetric"
  [sda_QuadraticCalc_p3] -> MetricCompare/2(quadraticMetric)
  [sda_QuadraticCalc_p3] -> BranchMemory/8(quadraticMetric)
  [sda_QuadraticCalc_p3] -> DebugBusCreator/6
  QuadraticCalc/4(head) -> [sda_QuadraticCalc_p4]  "head"
  [sda_QuadraticCalc_p4] -> DebugBusCreator/4
  QuadraticCalc/5(center) -> [sda_QuadraticCalc_p5]  "center"
  [sda_QuadraticCalc_p5] -> DebugBusCreator/5
  QuadraticCalc/6(firstCandidate) -> QuadFirstCandidateTerminator/1
  QuadraticCalc/7(candidate) -> [sda_QuadraticCalc_p7]
  [sda_QuadraticCalc_p7] -> BranchMemory/7(candidate)
  [sda_QuadraticCalc_p7] -> QuadCandidateDelay/1
  QuadraticCalc/8(residual) -> QuadResidualTerminator/1
  VectorCostCalc/2(valid) -> [sda_VectorCostCalc_p2]
  [sda_VectorCostCalc_p2] -> StatusDelay6/1
  VectorCostCalc/3(totalMetricNew) -> [sda_VectorCostCalc_p3]  "vectorMetric"
  [sda_VectorCostCalc_p3] -> DebugBusCreator/7
  [sda_VectorCostCalc_p3] -> MetricCompare/3(vectorMetric)
  [sda_VectorCostCalc_p3] -> BranchMemory/9(vectorMetric)
  VectorCostCalc/4(cmvMetricNew) -> [sda_VectorCostCalc_p4]
  [sda_VectorCostCalc_p4] -> BranchMemory/10(cmvMetric)
  [sda_VectorCostCalc_p4] -> MetricCompare/4(vectorCmvMetric)
  VectorCostCalc/5(cmvIncrement) -> CmvIncrementTerminator/1
  VectorCostCalc/6(iabcNext) -> [sda_VectorCostCalc_p6]
  [sda_VectorCostCalc_p6] -> BranchMemory/11(iabcNext)
  VectorCostCalc/7(deltaStep) -> DeltaStepTerminator/1
  VectorCostCalc/8(deltaDead) -> DeltaDeadTerminator/1
  VectorCostCalc/9(lowerBound) -> LowerBoundTerminator/1
  VectorCostCalc/10(upperBound) -> UpperBoundTerminator/1
  VectorCostCalc/11(deadtimeMiss) -> DeadtimeMissTerminator/1
  BranchMemory/1(memory) -> BranchMemoryStateDelay/1
  BranchMemory/2(candidateExhausted) -> [sda_BranchMemory_p2]
  [sda_BranchMemory_p2] -> CandidateExhaustedDelay/1
  MetricCompare/3(better) -> [sda_MetricCompare_p3]
  [sda_MetricCompare_p3] -> MetricBetterDelay/1
  MetricCompare/4(prune) -> MetricPruneDelay/1
  [currentPrune] -> SearchFSM/11(currentPrune)
  [currentPrune] -> SearchCounter/6(currentPrune)
  LatchedIabcSelector/1 -> BranchMemory/13(iabcInitial)  "<iabcCompensated>"
  [sda_start_pulse] -> ProblemLatch/2(loadEnable)  "start_pulse"

== matlab function SDA_PL_Harness_2025b/PlaybackController ==
  data: busy input; caseIndex output; resultValid input; fault input; caseLimit input; start output; compareEnable output; done output
function [caseIndex,start,compareEnable,done] = fcn(busy,resultValid,fault,caseLimit)
%#codegen
persistent index state
if isempty(index), index=uint32(1); state=uint8(0); end
caseIndex=index; start=false; compareEnable=false; done=false;
switch state
 case 0 % allow selected problem to settle
  if caseLimit==0, done=true; else, state=uint8(1); end
 case 1 % exactly one 100 MHz start pulse
  start=true; state=uint8(2);
 case 2 % hold inputs while PL searches
  if fault, compareEnable=true; state=uint8(3);
  elseif resultValid, compareEnable=true; state=uint8(3); end
 case 3 % advance only after comparison sampled the old index
  if index>=caseLimit, done=true; state=uint8(4);
  else, index=index+uint32(1); state=uint8(0); end
 otherwise
  done=true;
end
end

== matlab function SDA_PL_Harness_2025b/SDA_PL_Framework/BestMemory ==
  data: initWrite input boolean size=[1 1]; searchWrite input boolean size=[1 1]; best output Bus: SdaBestBus size=[1 1]; initialU input double size=[15 1]; initialMetric input double size=[1 1]; initialCmv input double size=[1 1]; memory input Bus: SdaMemoryBus size=[1 1]; candidateMetric input double size=[1 1]; candidateCmv input double size=[1 1]
function best = BestMemory(initWrite,searchWrite,initialU,initialMetric,initialCmv,memory,candidateMetric,candidateCmv)
%#codegen
persistent state
if isempty(state)
 state.bestU=false(15,1); state.bestMetric=realmax;
 state.bestCMVCost=0.0; state.bestValid=false;
end
if initWrite
 state.bestU=initialU>0.5; state.bestMetric=initialMetric;
 state.bestCMVCost=initialCmv; state.bestValid=isfinite(initialMetric);
elseif searchWrite&&candidateMetric<state.bestMetric
 state.bestU=memory.Uwork; state.bestMetric=candidateMetric;
 state.bestCMVCost=candidateCmv; state.bestValid=isfinite(candidateMetric);
end
best=state;
end

== matlab function SDA_PL_Harness_2025b/SDA_PL_Framework/BranchMemory ==
  data: clear input boolean size=[1 1]; initWrite input boolean size=[1 1]; memory output Bus: SdaMemoryBus size=[1 1]; pathWrite input boolean size=[1 1]; vectorWrite input boolean size=[1 1]; level input uint8 size=[1 1]; fsmState input uint8 size=[1 1]; candidate input boolean size=[1 1]; quadraticMetric input double size=[1 1]; vectorMetric input double size=[1 1]; cmvMetric input double size=[1 1]; iabcNext input double size=[3 1]; z input double size=[15 1]; iabcInitial input double size=[3 1]; candidateExhausted output boolean size=[1 1]
function [memory,candidateExhausted] = BranchMemory(clear,initWrite,pathWrite,vectorWrite,level,fsmState,candidate,quadraticMetric,vectorMetric,cmvMetric,iabcNext,z,iabcInitial)
%#codegen
persistent state
if isempty(state)
    state.Uwork=false(15,1);
    state.candidatePosition=ones(15,1,'uint8');
    state.metricStack=zeros(16,1); state.cmvMetricStack=zeros(16,1);
    state.iabcPrediction=zeros(3,6); state.z=zeros(15,1);
end
idx=max(uint8(1),min(uint8(15),level));
if clear
    state.Uwork(:)=false; state.candidatePosition(:)=uint8(1);
    state.metricStack(:)=0.0; state.cmvMetricStack(:)=0.0;
    state.iabcPrediction(:)=0.0; state.z(:)=0.0;
end
if initWrite
    state.z=z; state.iabcPrediction(:,1)=iabcInitial;
    state.metricStack(1)=0.0; state.cmvMetricStack(1)=0.0;
end
if pathWrite
    if fsmState==uint8(7)
        state.Uwork(idx)=candidate;
        state.candidatePosition(idx)=state.candidatePosition(idx)+uint8(1);
        state.metricStack(double(idx)+1)=quadraticMetric;
        state.cmvMetricStack(double(idx)+1)=state.cmvMetricStack(double(idx));
    elseif fsmState==uint8(15)
        state.candidatePosition(idx)=uint8(1);
    elseif fsmState==uint8(17)
        resetIdx=min(uint8(15),idx+uint8(1));
        state.candidatePosition(resetIdx)=uint8(1);
    end
end
if vectorWrite
    state.metricStack(double(idx)+1)=vectorMetric;
    state.cmvMetricStack(double(idx)+1)=cmvMetric;
    predictionStep=idivide(idx,uint8(3));
    currentColumn=min(6,double(predictionStep)+1);
    state.iabcPrediction(:,currentColumn)=iabcNext;
end
candidateExhausted=state.candidatePosition(idx)>uint8(2);
memory=state;
end

== matlab function SDA_PL_Harness_2025b/SDA_PL_Framework/MetricCompare ==
  data: level input uint8 size=[1 1]; currentMetric output double size=[1 1]; quadraticMetric input double size=[1 1]; vectorMetric input double size=[1 1]; vectorCmvMetric input double size=[1 1]; memory input Bus: SdaMemoryBus size=[1 1]; best input Bus: SdaBestBus size=[1 1]; currentCmvMetric output double size=[1 1]; better output boolean size=[1 1]; prune output boolean size=[1 1]
function [currentMetric,currentCmvMetric,better,prune] = MetricCompare(level,quadraticMetric,vectorMetric,vectorCmvMetric,memory,best)
%#codegen
idx=max(uint8(1),min(uint8(15),level));
if mod(idx,uint8(3))==uint8(0)
 currentMetric=vectorMetric; currentCmvMetric=vectorCmvMetric;
else
 currentMetric=quadraticMetric;
 currentCmvMetric=memory.cmvMetricStack(double(idx)+1);
end
better=currentMetric<best.bestMetric;
prune=currentMetric>best.bestMetric;
end

== matlab function SDA_PL_Harness_2025b/SDA_PL_Framework/ProblemLatch ==
  data: problemIn input Bus: SdaProblemBus size=[1 1]; problem output Bus: SdaProblemBus size=[1 1]; loadEnable input boolean size=[1 1]
function problem = ProblemLatch(problemIn, loadEnable)
%#codegen
persistent latchedProblem
if isempty(latchedProblem)
    latchedProblem = problemIn;
end
if loadEnable
    latchedProblem = problemIn;
end
problem = latchedProblem;

== matlab function SDA_PL_Harness_2025b/SDA_PL_Framework/QuadraticCalc ==
  data: problem input Bus: SdaProblemBus size=[1 1]; done output boolean size=[1 1]; start input boolean size=[1 1]; level input uint8 size=[1 1]; memory input Bus: SdaMemoryBus size=[1 1]; valid output boolean size=[1 1]; metricNew output double size=[1 1]; head output double size=[1 1]; center output double size=[1 1]; firstCandidate output boolean size=[1 1]; candidate output boolean size=[1 1]; residual output double size=[1 1]
function [done, valid, metricNew, head, center, firstCandidate, candidate, residual] = QuadraticCalc(problem, start, level, memory)
%#codegen
persistent metricReg headReg centerReg firstReg candidateReg residualReg validReg
if isempty(metricReg)
    metricReg=0.0; headReg=0.0; centerReg=0.0;
    firstReg=false; candidateReg=false; residualReg=0.0; validReg=false;
end
done=false;
if start
    idx=max(uint8(1),min(uint8(15),level));
    row=double(idx); headReg=0.0;
    for k=1:15
        if k<row
            headReg=headReg+problem.H(row,k)*double(memory.Uwork(k));
        end
    end
    diagonal=problem.H(row,row);
    validReg=isfinite(diagonal)&&abs(diagonal)>1e-12;
    if validReg
        centerReg=(memory.z(row)-headReg)/diagonal;
        firstReg=centerReg>0.5;
        if memory.candidatePosition(row)==uint8(1)
            candidateReg=firstReg;
        else
            candidateReg=~firstReg;
        end
        residualReg=memory.z(row)-headReg-diagonal*double(candidateReg);
        metricReg=memory.metricStack(row)+residualReg*residualReg;
        validReg=isfinite(centerReg)&&isfinite(metricReg);
    else
        centerReg=0.0; firstReg=false; candidateReg=false;
        residualReg=0.0; metricReg=realmax;
    end
    done=true;
end
valid=validReg; metricNew=metricReg; head=headReg; center=centerReg;
firstCandidate=firstReg; candidate=candidateReg; residual=residualReg;
end

== matlab function SDA_PL_Harness_2025b/SDA_PL_Framework/ResultCommit ==
  data: problem input Bus: SdaProblemBus size=[1 1]; result output Bus: SdaResultBus size=[1 1]; commit input boolean size=[1 1]; best input Bus: SdaBestBus size=[1 1]; nodes input uint32 size=[1 1]; leafNodes input uint32 size=[1 1]; nodeLimitReached input boolean size=[1 1]; Jround input double size=[1 1]; Jshift input double size=[1 1]
function result = ResultCommit(problem,commit,best,nodes,leafNodes,nodeLimitReached,Jround,Jshift)
%#codegen
persistent state
if isempty(state)
 state.valid=false; state.Jopt=realmax; state.nodes=uint32(0);
 state.optimal=false; state.Uopt=zeros(15,1); state.Uapply=zeros(6,1);
 state.leafNodes=uint32(0); state.bestCMVCost=0.0; state.cmvMetricRatio=0.0;
 state.switchCountApplied=uint32(0); state.debugLower=zeros(3,1);
 state.debugUpper=zeros(3,1); state.iabcPredictedNext=zeros(3,1);
 state.Jround=0.0; state.Jshift=0.0; state.predictionValidNext=false; state.solutionToggle=false;
end
if commit
 state.valid=best.bestValid; state.Jopt=best.bestMetric;
 state.nodes=nodes; state.leafNodes=leafNodes;
 state.optimal=best.bestValid&&~nodeLimitReached;
 state.Uopt=double(best.bestU); state.Uapply=state.Uopt(1:6);
 state.bestCMVCost=best.bestCMVCost;
 if state.Jopt>eps, state.cmvMetricRatio=state.bestCMVCost/state.Jopt; else, state.cmvMetricRatio=0.0; end
 sPrev=problem.UoptPrev(4:6); sFirst=state.Uopt(1:3); sSecond=state.Uopt(4:6);
 [deltaFirst,deltaDead]=deadtime_step(sPrev,sFirst,problem.iabcCompensated,problem);
 iabcAfter=problem.iabcCompensated+deltaFirst;
 [deltaSecond,~]=deadtime_step(sFirst,sSecond,iabcAfter,problem);
 state.iabcPredictedNext=iabcAfter+deltaSecond;
 state.switchCountApplied=uint32(sum(abs(sFirst-sPrev))+sum(abs(sSecond-sFirst)));
 [~,state.debugLower,state.debugUpper]=cmv_bounds(problem.iabcCompensated,deltaDead,problem.currentEpsMargin);
 state.Jround=Jround; state.Jshift=Jshift; state.predictionValidNext=best.bestValid;
 state.solutionToggle=~state.solutionToggle;
end
result=state;
end

function [deltaStep,deltaDead]=deadtime_step(sPrevious,sCurrent,iabc,problem)
sDead=sCurrent; signEps=0.1*problem.currentEpsMargin;
for phase=1:3
 if sPrevious(phase)~=sCurrent(phase)
  if iabc(phase)>=signEps, sDead(phase)=0.0;
  elseif iabc(phase)<=-signEps, sDead(phase)=1.0;
  elseif signEps>0.0, sDead(phase)=0.5*(1.0-iabc(phase)/signEps);
  else, sDead(phase)=0.5; end
 end
end
sEffective=problem.deadtimeRatio*sDead+(1.0-problem.deadtimeRatio)*sCurrent;
deltaDead=problem.deadtimeRatio*(problem.deltaIabcBase+problem.deltaIabcSwitch*sDead);
deltaStep=problem.deltaIabcBase+problem.deltaIabcSwitch*sEffective;
end

function [iabcEnd,lower,upper]=cmv_bounds(iabc,deltaDead,margin)
iabcEnd=iabc+deltaDead; lower=min(iabc,iabcEnd)-margin; upper=max(iabc,iabcEnd)+margin;
end

== matlab function SDA_PL_Harness_2025b/SDA_PL_Framework/SdaInitializer ==
  data: problem input Bus: SdaProblemBus size=[1 1]; done output boolean size=[1 1]; start input boolean size=[1 1]; valid output boolean size=[1 1]; z output double size=[15 1]; initialU output double size=[15 1]; initialMetric output double size=[1 1]; initialCMVCost output double size=[1 1]; Jround output double size=[1 1]; Jshift output double size=[1 1]
function [done, valid, z, initialU, initialMetric, initialCMVCost, Jround, Jshift] = SdaInitializer(problem, start)
%#codegen
persistent zReg uReg metricReg cmvReg jRoundReg jShiftReg validReg
if isempty(zReg)
    zReg=zeros(15,1); uReg=zeros(15,1); metricReg=realmax;
    cmvReg=0.0; jRoundReg=0.0; jShiftReg=0.0; validReg=false;
end
done=false;
if start
    zReg=problem.H*problem.U_unc;
    uRound=zeros(15,1); uShift=zeros(15,1);
    for k=1:15
        uRound(k)=min(max(round(problem.U_unc(k)),0.0),1.0);
    end
    for k=1:12
        uShift(k)=problem.UoptPrev(k+3);
    end
    for k=13:15
        uShift(k)=problem.UoptPrev(k);
    end
    jRoundReg=quadratic_cost(problem.H,uRound,problem.U_unc);
    jShiftReg=quadratic_cost(problem.H,uShift,problem.U_unc);
    if jShiftReg < jRoundReg
        uReg=uShift;
    else
        uReg=uRound;
    end
    sPrevious=problem.UoptPrev(4:6);
    cmvReg=sequence_cmv_cost(uReg,sPrevious,problem);
    metricReg=quadratic_cost(problem.H,uReg,problem.U_unc)+cmvReg;
    validReg=isfinite(metricReg);
    done=true;
end
valid=validReg; z=zReg; initialU=uReg; initialMetric=metricReg;
initialCMVCost=cmvReg; Jround=jRoundReg; Jshift=jShiftReg;
end

function value=quadratic_cost(H,U,Uunc)
residual=H*(U-Uunc);
value=norm(residual,2)^2;
end

function total=sequence_cmv_cost(U,sPrevious,problem)
total=0.0; iabc=problem.iabcCompensated;
for step=1:5
    first=(step-1)*3+1; sCurrent=U(first:first+2);
    [deltaStep,deltaDead]=deadtime_step(sPrevious,sCurrent,iabc,problem);
    total=total+cmv_penalty(sPrevious,sCurrent,iabc,deltaDead,problem);
    iabc=iabc+deltaStep; sPrevious=sCurrent;
end
end

function [deltaStep,deltaDead]=deadtime_step(sPrevious,sCurrent,iabc,problem)
sDead=sCurrent; signEps=0.1*problem.currentEpsMargin;
for phase=1:3
    if sPrevious(phase)~=sCurrent(phase)
        if iabc(phase)>=signEps
            sDead(phase)=0.0;
        elseif iabc(phase)<=-signEps
            sDead(phase)=1.0;
        elseif signEps>0.0
            sDead(phase)=0.5*(1.0-iabc(phase)/signEps);
        else
            sDead(phase)=0.5;
        end
    end
end
sEffective=problem.deadtimeRatio*sDead+(1.0-problem.deadtimeRatio)*sCurrent;
deltaDead=problem.deadtimeRatio*(problem.deltaIabcBase+problem.deltaIabcSwitch*sDead);
deltaStep=problem.deltaIabcBase+problem.deltaIabcSwitch*sEffective;
end

function penalty=cmv_penalty(sPrevious,sCurrent,iabc,deltaDead,problem)
penalty=0.0; iabcEnd=iabc+deltaDead;
lower=min(iabc,iabcEnd)-problem.currentEpsMargin;
upper=max(iabc,iabcEnd)+problem.currentEpsMargin;
uncertain=(lower<=0.0)&(upper>=0.0);
if all(sCurrent==0.0)||all(sCurrent==1.0)
    penalty=penalty+problem.lambdaZero;
end
changed=(sPrevious~=sCurrent);
if sum(changed)~=2
    return;
end
canZero=false(3,1); canOne=false(3,1);
for phase=1:3
    if ~changed(phase)
        canZero(phase)=sPrevious(phase)==0.0;
        canOne(phase)=sPrevious(phase)==1.0;
    elseif uncertain(phase)
        canZero(phase)=true; canOne(phase)=true;
    elseif iabcEnd(phase)>0.0
        canZero(phase)=true;
    else
        canOne(phase)=true;
    end
end
if all(canZero)||all(canOne)
    penalty=penalty+problem.lambdaDeadtime;
end
end

== matlab function SDA_PL_Harness_2025b/SDA_PL_Framework/SearchCounter ==
  data: clear input boolean size=[1 1]; nodes output uint32 size=[1 1]; writeEnable input boolean size=[1 1]; fsmState input uint8 size=[1 1]; level input uint8 size=[1 1]; problem input Bus: SdaProblemBus size=[1 1]; leafNodes output uint32 size=[1 1]; nodeLimitReached output boolean size=[1 1]; currentPrune input boolean size=[1 1]
function [nodes,leafNodes,nodeLimitReached] = SearchCounter(clear,writeEnable,fsmState,level,problem,currentPrune)
%#codegen
persistent nodeReg leafReg limitReg leafStatePrev
if isempty(nodeReg), nodeReg=uint32(0); leafReg=uint32(0); limitReg=false; leafStatePrev=false; end
if clear, nodeReg=uint32(0); leafReg=uint32(0); limitReg=false; leafStatePrev=false; end
if writeEnable&&fsmState==uint8(7)
 nodeReg=nodeReg+uint32(1);
 if problem.NmaxNode>uint32(0)&&nodeReg>problem.NmaxNode, limitReg=true; end
end
leafStateNow=fsmState==uint8(16);
if leafStateNow&&~leafStatePrev&&level==uint8(15)&&~currentPrune
 leafReg=leafReg+uint32(1);
end
leafStatePrev=leafStateNow;
nodes=nodeReg; leafNodes=leafReg; nodeLimitReached=limitReg;
end
